simulink model "fifth_lab"  (R2025b)
settings: Solver=VariableStepAuto  StartTime=0.0  StopTime=10.0  RelTol=1e-3
values from neighbouring files (symbols this model uses):
  dx0 = 0    [lab5.m]
  x0 = pi/2    (= 1.57079632679)    [lab5.m]
settings Model: Creator=reino  LastModifiedBy=reino

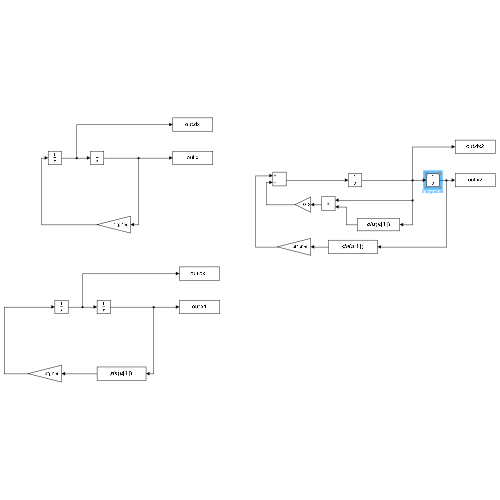
[thumbnail: Simulink's stored preview of the top-level diagram]
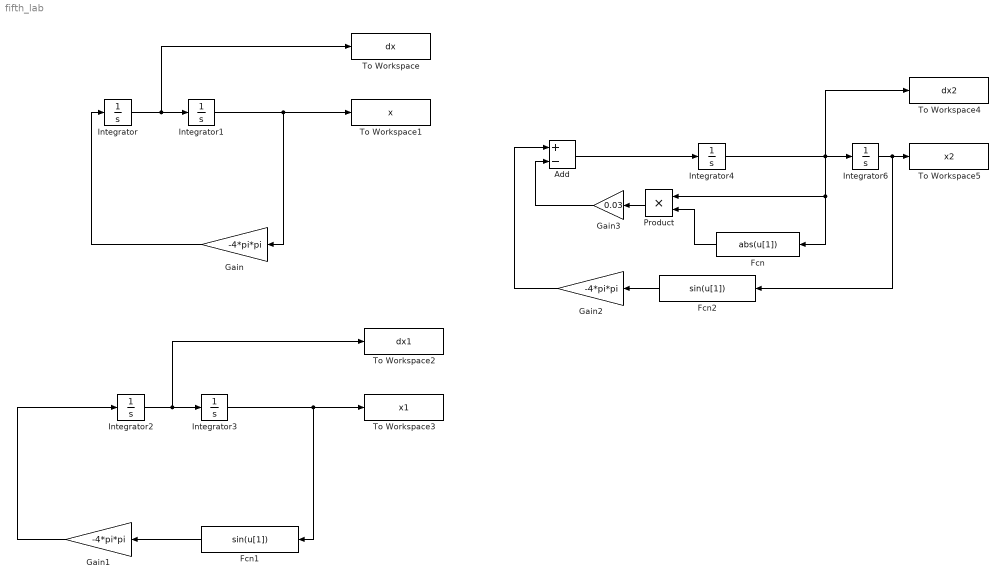
== system fifth_lab ==
  Add : Sum  Inputs=+-
  Fcn : Fcn  Expr=abs(u[1])
  Fcn1 : Fcn
  Fcn2 : Fcn
  Gain : Gain  Gain=-4*pi*pi
  Gain1 : Gain  Gain=-4*pi*pi
  Gain2 : Gain  Gain=-4*pi*pi
  Gain3 : Gain  Gain=0.03
  Integrator : Integrator  InitialCondition=x0
  Integrator1 : Integrator  InitialCondition=dx0
  Integrator2 : Integrator  InitialCondition=x0
  Integrator3 : Integrator  InitialCondition=dx0
  Integrator4 : Integrator  InitialCondition=x0
  Integrator6 : Integrator  InitialCondition=dx0
  Product : Product
  To Workspace : ToWorkspace  VariableName=dx  SampleTime=-1
  To Workspace1 : ToWorkspace  VariableName=x  SampleTime=-1
  To Workspace2 : ToWorkspace  VariableName=dx1  SampleTime=-1
  To Workspace3 : ToWorkspace  VariableName=x1  SampleTime=-1
  To Workspace4 : ToWorkspace  VariableName=dx2  SampleTime=-1
  To Workspace5 : ToWorkspace  VariableName=x2  SampleTime=-1
  wires:
  Integrator1/1 -> Gain/1, To Workspace1/1
  Integrator/1 -> To Workspace/1, Integrator1/1
  Gain/1 -> Integrator/1
  Fcn1/1 -> Gain1/1
  Integrator3/1 -> Fcn1/1, To Workspace3/1
  Integrator2/1 -> To Workspace2/1, Integrator3/1
  Gain1/1 -> Integrator2/1
  Fcn2/1 -> Gain2/1
  Integrator6/1 -> Fcn2/1, To Workspace5/1
  Integrator4/1 -> To Workspace4/1, Fcn/1, Product/1, Integrator6/1
  Fcn/1 -> Product/2
  Product/1 -> Gain3/1
  Add/1 -> Integrator4/1
  Gain3/1 -> Add/2
  Gain2/1 -> Add/1
